simulink model "SimBasZEnvioTodo"  (R2026b)
settings: Solver=VariableStepAuto  StopTime=inf
undefined symbols (not defined in the file): heartbeatBytes, Payload, SampleTime
libraries: uavmavlinklib x8, simulink x1, sharedtransform x1
settings Model: Creator=cfmm  LastModifiedBy=cfmm

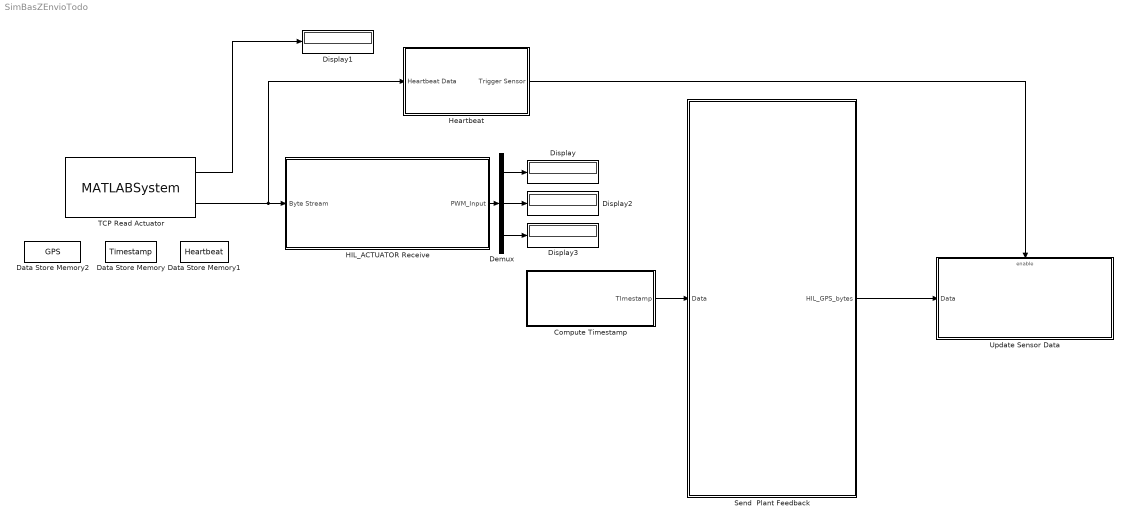
== system SimBasZEnvioTodo ==
  Compute Timestamp : Subsystem
  Data Store Memory : DataStoreMemory  DataStoreName=Timestamp  WriteAfterWriteMsg=warning  ShowAdditionalParam=off
  Data Store Memory1 : DataStoreMemory  DataStoreName=Heartbeat  WriteAfterWriteMsg=warning  InitialValue=1  ShowAdditionalParam=off
  Data Store Memory2 : DataStoreMemory  DataStoreName=GPS  WriteAfterWriteMsg=warning  ShowAdditionalParam=off
  Demux : Demux  Outputs=3
  Display{,1..3} (4 alike) : Display
  HIL_ACTUATOR Receive : Subsystem
  Heartbeat : Subsystem
  Send  Plant Feedback : Subsystem
  TCP Read Actuator : MATLABSystem  System=px4HostTarget_TCPIP_Read  Length=actuatorBytes  SampleTime=SampleTime
      mask Type: px4HostTarget_TCPIP_Read
  "Update Sensor Data " : Subsystem
  wires:
  TCP Read Actuator/1 -> Display1/1
  TCP Read Actuator/2 -> Heartbeat/1(Heartbeat Data), HIL_ACTUATOR Receive/1(Byte Stream)
  Send  Plant Feedback/1(HIL_GPS_bytes) -> "Update Sensor Data "/1(Data)
  Heartbeat/1(Trigger Sensor) -> "Update Sensor Data "/Enable
  HIL_ACTUATOR Receive/1(PWM_Input) -> Demux/1
  Demux/1 -> Display/1
  Demux/2 -> Display2/1
  Demux/3 -> Display3/1
  Compute Timestamp/1(TImestamp) -> Send  Plant Feedback/1(Data)

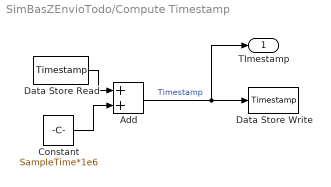
== system SimBasZEnvioTodo/Compute Timestamp ==
  Add : Sum
  Constant : Constant  Value=SampleTime*1e6  OutDataTypeStr=uint64  SampleTime=SampleTime
  Data Store Read : DataStoreRead  DataStoreName=Timestamp  SampleTime=SampleTime  IndexOptions=Index vector (dialog)  Indices=1  OutputSizes=1
  Data Store Write : DataStoreWrite  DataStoreName=Timestamp  SampleTime=SampleTime  IndexOptions=Index vector (dialog)  Indices=1  OutputSizes=1
  TImestamp : Outport
  wires:
  Data Store Read/1 -> Add/1
  Add/1 -> TImestamp/1, Data Store Write/1  "Timestamp"
  Constant/1 -> Add/2

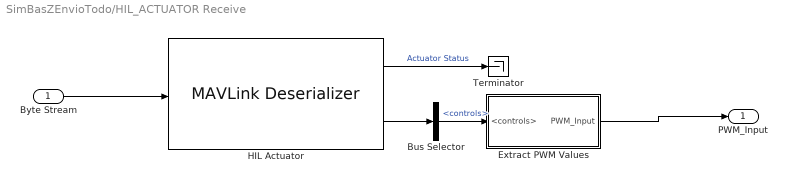
== system SimBasZEnvioTodo/HIL_ACTUATOR Receive ==
  Byte Stream : Inport
  Bus Selector : BusSelector  OutputSignals=Payload.controls
  Extract PWM Values : Subsystem
  HIL Actuator : uavmavlinklib/MAVLink Deserializer  dialectSource=Select from standard MAVLink dialects  dialect=common.xml  dialectCustom=common.xml  version=2  messageType=HIL_ACTUATOR_CONTROLS  inputDataLength=off  SystemIDFilter=off  systemID=1  ComponentIDFilter=off  componentID=1  queueMsg=off  queueMsgSize=50  dropNum=off
  Terminator : Terminator
  PWM_Input : Outport
  wires:
  Byte Stream/1 -> HIL Actuator/1
  HIL Actuator/2 -> Bus Selector/1
  Bus Selector/1 -> Extract PWM Values/1(<controls>)  "<controls>"
  Extract PWM Values/1(PWM_Input) -> PWM_Input/1
  HIL Actuator/1 -> Terminator/1  "Actuator Status"

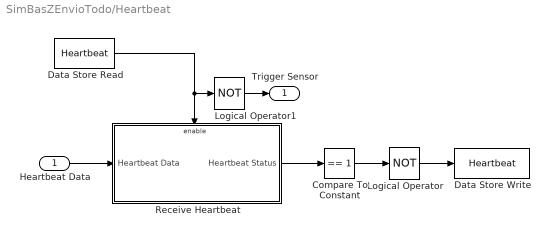
== system SimBasZEnvioTodo/Heartbeat ==
  Heartbeat Data : Inport
  Compare To Constant : simulink/Logic and Bit Operations/Compare To Constant  relop===  const=1  OutDataTypeStr=uint8
  Data Store Read : DataStoreRead  DataStoreName=Heartbeat  SampleTime=SampleTime  IndexOptions=Index vector (dialog)  Indices=1  OutputSizes=1
  Data Store Write : DataStoreWrite  DataStoreName=Heartbeat  SampleTime=SampleTime  IndexOptions=Index vector (dialog)  Indices=1  OutputSizes=1
  Logical Operator : Logic  Operator=NOT  AllPortsSameDT=off  OutDataTypeStr=boolean
  Logical Operator1 : Logic  Operator=NOT  AllPortsSameDT=off  OutDataTypeStr=boolean
  Receive Heartbeat : Subsystem
  Trigger Sensor : Outport
  wires:
  Logical Operator/1 -> Data Store Write/1
  Data Store Read/1 -> Receive Heartbeat/Enable, Logical Operator1/1
  Receive Heartbeat/1(Heartbeat Status) -> Compare To Constant/1
  Compare To Constant/1 -> Logical Operator/1
  Heartbeat Data/1 -> Receive Heartbeat/1(Heartbeat Data)
  Logical Operator1/1 -> Trigger Sensor/1

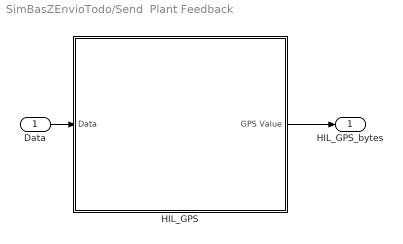
== system SimBasZEnvioTodo/Send  Plant Feedback ==
  Data : Inport
  HIL_GPS : Subsystem
  HIL_GPS_bytes : Outport
  wires:
  HIL_GPS/1(GPS Value) -> HIL_GPS_bytes/1
  Data/1 -> HIL_GPS/1(Data)

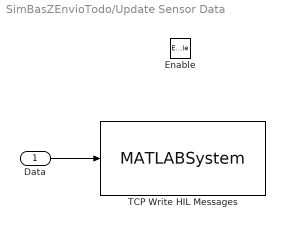
== system SimBasZEnvioTodo/Update Sensor Data  ==
  Data : Inport
  Enable : EnablePort
  TCP Write HIL Messages : MATLABSystem  System=px4HostTarget_TCPIP_Write
      mask Type: px4HostTarget_TCPIP_Write
  wires:
  Data/1 -> TCP Write HIL Messages/1

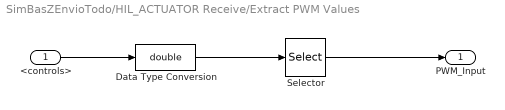
== system SimBasZEnvioTodo/HIL_ACTUATOR Receive/Extract PWM Values ==
  <controls> : Inport
  Data Type Conversion : DataTypeConversion  OutDataTypeStr=double  SaturateOnIntegerOverflow=off  RndMeth=Floor
  Selector : Selector  InputPortWidth=16  IndexOptions=Index vector (dialog)  Indices=[1:3]  OutputSizes=1  RuntimeRangeChecks=off
  PWM_Input : Outport
  wires:
  Data Type Conversion/1 -> Selector/1
  <controls>/1 -> Data Type Conversion/1
  Selector/1 -> PWM_Input/1

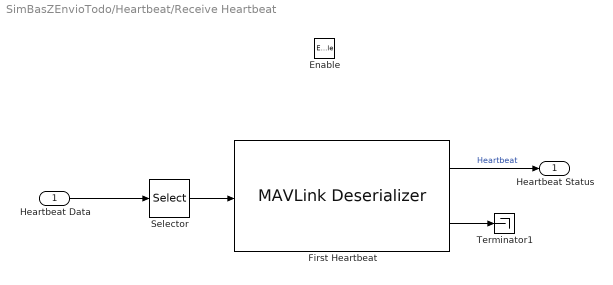
== system SimBasZEnvioTodo/Heartbeat/Receive Heartbeat ==
  Heartbeat Data : Inport
  Enable : EnablePort
  First Heartbeat : uavmavlinklib/MAVLink Deserializer  dialectSource=Select from standard MAVLink dialects  dialect=common.xml  dialectCustom=common.xml  version=2  messageType=HEARTBEAT  inputDataLength=off  SystemIDFilter=off  systemID=1  ComponentIDFilter=off  componentID=1  queueMsg=off  queueMsgSize=50  dropNum=off
  Selector : Selector  InputPortWidth=93  IndexOptions=Index vector (dialog)  Indices=[1:heartbeatBytes]  OutputSizes=1  RuntimeRangeChecks=off
  Terminator1 : Terminator
  Heartbeat Status : Outport
  wires:
  First Heartbeat/2 -> Terminator1/1
  Selector/1 -> First Heartbeat/1
  First Heartbeat/1 -> Heartbeat Status/1  "Heartbeat"
  Heartbeat Data/1 -> Selector/1

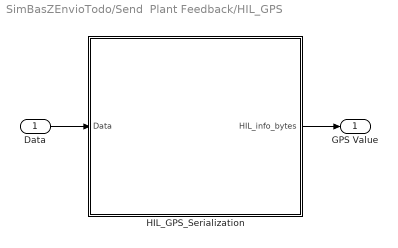
== system SimBasZEnvioTodo/Send  Plant Feedback/HIL_GPS ==
  Data : Inport
  HIL_GPS_Serialization : Subsystem
  GPS Value : Outport
  wires:
  HIL_GPS_Serialization/1(HIL_info_bytes) -> GPS Value/1
  Data/1 -> HIL_GPS_Serialization/1(Data)

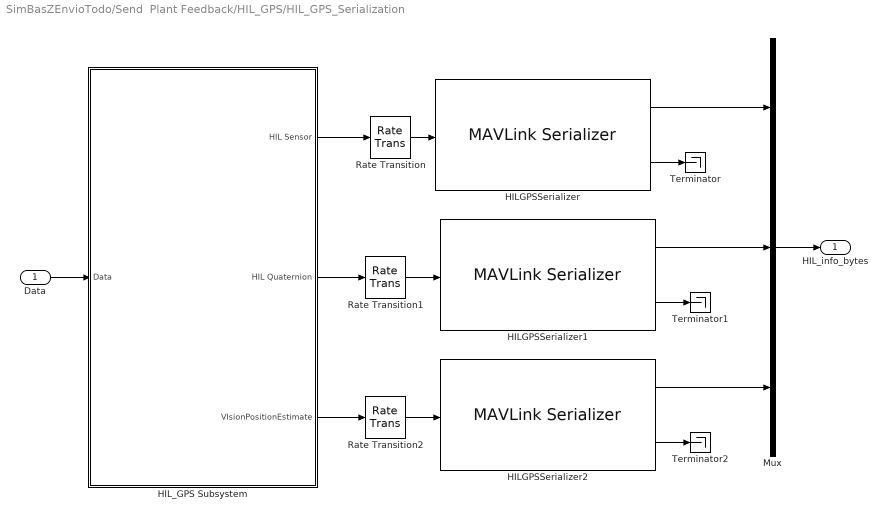
== system SimBasZEnvioTodo/Send  Plant Feedback/HIL_GPS/HIL_GPS_Serialization ==
  Data : Inport
  HILGPSSerializer : uavmavlinklib/MAVLink Serializer  dialectSource=Select from standard MAVLink dialects  dialect=common.xml  dialectCustom=common.xml  version=2  messageType=HIL_SENSOR
  HILGPSSerializer1 : uavmavlinklib/MAVLink Serializer  dialectSource=Select from standard MAVLink dialects  dialect=common.xml  dialectCustom=common.xml  version=2  messageType=HIL_STATE_QUATERNION
  HILGPSSerializer2 : uavmavlinklib/MAVLink Serializer  dialectSource=Select from standard MAVLink dialects  dialect=common.xml  dialectCustom=common.xml  version=2  messageType=VISION_POSITION_ESTIMATE
  HIL_GPS Subsystem : Subsystem
  Mux : Mux  Inputs=3
  Rate Transition : RateTransition  OutPortSampleTime=SampleTime
  Rate Transition1 : RateTransition  OutPortSampleTime=SampleTime
  Rate Transition2 : RateTransition  OutPortSampleTime=SampleTime
  Terminator : Terminator
  Terminator1 : Terminator
  Terminator2 : Terminator
  HIL_info_bytes : Outport
  wires:
  HILGPSSerializer/2 -> Terminator/1
  HIL_GPS Subsystem/1(HIL Sensor) -> Rate Transition/1
  Rate Transition/1 -> HILGPSSerializer/1
  Rate Transition1/1 -> HILGPSSerializer1/1
  HILGPSSerializer1/2 -> Terminator1/1
  HILGPSSerializer2/1 -> Mux/3
  Rate Transition2/1 -> HILGPSSerializer2/1
  HILGPSSerializer2/2 -> Terminator2/1
  HIL_GPS Subsystem/2(HIL Quaternion) -> Rate Transition1/1
  HIL_GPS Subsystem/3(VIsionPositionEstimate) -> Rate Transition2/1
  HILGPSSerializer/1 -> Mux/1
  HILGPSSerializer1/1 -> Mux/2
  Mux/1 -> HIL_info_bytes/1
  Data/1 -> HIL_GPS Subsystem/1(Data)

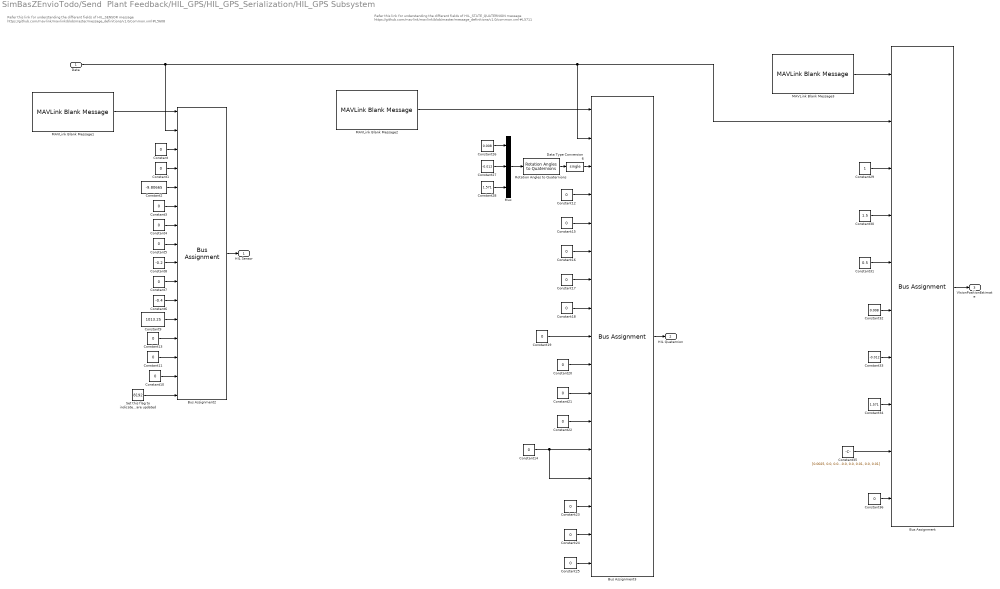
== system SimBasZEnvioTodo/Send  Plant Feedback/HIL_GPS/HIL_GPS_Serialization/HIL_GPS Subsystem ==
  note: Refer this link for understanding the different fields of HIL_SENSOR message https://github.com/mavlink/mavlink/blob/master/message_definitions/v1.0/common.xml#L5608
  note: Refer this link for understanding the different fields of HIL_STATE_QUATERNION message https://github.com/mavlink/mavlink/blob/master/message_definitions/v1.0/common.xml#L5711
  Data : Inport
  Bus Assignment : BusAssignment  AssignedSignals=Payload.usec,Payload.x,Payload.y,Payload.z,Payload.roll,Payload.pitch,Payload.yaw,Payload.covariance,Payload.reset_counter
  Bus Assignment2 : BusAssignment  AssignedSignals=Payload.time_usec,Payload.xacc,Payload.yacc,Payload.zacc,Payload.xgyro,Payload.ygyro,Payload.zgyro,Payload.xmag,Payload.ymag,Payload.zmag,Payload.abs_pressure,Payload.diff_pressure,Payload.pressure_alt,Payload.temperature,Payload.fields_updated
  Bus Assignment3 : BusAssignment  AssignedSignals=Payload.time_usec,Payload.attitude_quaternion,Payload.rollspeed,Payload.pitchspeed,Payload.yawspeed,Payload.lat,Payload.lon,Payload.alt,Payload.vx,Payload.vy,Payload.vz,Payload.ind_airspeed,Payload.true_airspeed,Payload.xacc,Payload.yacc,Payload.zacc
  Constant{,1,3..5,7} (6 alike) : Constant  Value=0  OutDataTypeStr=single
  Constant{10..13,15..16} (6 alike) : Constant  Value=0  OutDataTypeStr=single  SampleTime=SampleTime
  Constant14 : Constant  Value=0  OutDataTypeStr=Inherit: Inherit via back propagation
  Constant17 : Constant  Value=0  OutDataTypeStr=int32  SampleTime=SampleTime
  Constant18 : Constant  Value=0  OutDataTypeStr=int32  SampleTime=SampleTime
  Constant19 : Constant  Value=0  OutDataTypeStr=int32  SampleTime=SampleTime
  Constant2 : Constant  Value=-9.80665  OutDataTypeStr=single
  Constant{20..25} (6 alike) : Constant  Value=0  OutDataTypeStr=int16  SampleTime=SampleTime
  Constant26 : Constant  Value=0.008  OutDataTypeStr=single  SampleTime=SampleTime
  Constant27 : Constant  Value=-0.012  OutDataTypeStr=single  SampleTime=SampleTime
  Constant28 : Constant  Value=1.571  OutDataTypeStr=single  SampleTime=SampleTime
  Constant29 : Constant  OutDataTypeStr=single  SampleTime=SampleTime
  Constant30 : Constant  Value=1.5  OutDataTypeStr=single  SampleTime=SampleTime
  Constant31 : Constant  Value=0.5  OutDataTypeStr=single  SampleTime=SampleTime
  Constant32 : Constant  Value=0.008  OutDataTypeStr=single  SampleTime=SampleTime
  Constant33 : Constant  Value=-0.012  OutDataTypeStr=single  SampleTime=SampleTime
  Constant34 : Constant  Value=1.571  OutDataTypeStr=single  SampleTime=SampleTime
  Constant35 : Constant  Value=[0.0025, 0.0, 0.0, 0.0, 0.0, 0.0, 0.0025, 0.0, 0.0, 0.0, 0.0, 0.0025, 0.0, 0.0, 0.0, 0.01, 0.0, 0.0, 0.01, 0.0, 0.01]  OutDataTypeStr=single  SampleTime=SampleTime
  Constant36 : Constant  Value=0  OutDataTypeStr=uint8  SampleTime=SampleTime
  Constant6 : Constant  Value=-0.4  OutDataTypeStr=single
  Constant8 : Constant  Value=-0.2  OutDataTypeStr=single
  Constant9 : Constant  Value=1013.25  OutDataTypeStr=single
  Data Type Conversion6 : DataTypeConversion  OutDataTypeStr=single  SaturateOnIntegerOverflow=off  RndMeth=Floor
  MAVLink Blank Message1 : uavmavlinklib/MAVLink Blank Message  dialectSource=Select from standard MAVLink dialects  dialect=common.xml  dialectCustom=common.xml  version=2  messageType=HIL_SENSOR  SystemID=2  ComponentID=51  SampleTime=SampleTime
  MAVLink Blank Message2 : uavmavlinklib/MAVLink Blank Message  dialectSource=Select from standard MAVLink dialects  dialect=common.xml  dialectCustom=common.xml  version=2  messageType=HIL_STATE_QUATERNION  SystemID=2  ComponentID=51  SampleTime=SampleTime
  MAVLink Blank Message3 : uavmavlinklib/MAVLink Blank Message  dialectSource=Select from standard MAVLink dialects  dialect=common.xml  dialectCustom=common.xml  version=2  messageType=VISION_POSITION_ESTIMATE  SystemID=2  ComponentID=51  SampleTime=SampleTime
  Mux : Mux  Inputs=3
  Rotation Angles to Quaternions : sharedtransform/Rotation Angles to Quaternions  rotationOrder=ZYX  aMode=aMode
  Set this flag to indicate all flags are updated : Constant  Value=8192  OutDataTypeStr=Inherit: Inherit via back propagation  SampleTime=SampleTime
  HIL Sensor : Outport
  HIL Quaternion : Outport  Port=2
  VIsionPositionEstimate : Outport  Port=3
  wires:
  MAVLink Blank Message1/1 -> Bus Assignment2/1
  Set this flag to indicate all flags are updated/1 -> Bus Assignment2/16
  Bus Assignment2/1 -> HIL Sensor/1
  Constant13/1 -> Bus Assignment2/13
  MAVLink Blank Message2/1 -> Bus Assignment3/1
  Constant14/1 -> Bus Assignment3/14, Bus Assignment3/13
  Rotation Angles to Quaternions/1 -> Data Type Conversion6/1
  Data Type Conversion6/1 -> Bus Assignment3/3
  Bus Assignment3/1 -> HIL Quaternion/1
  MAVLink Blank Message3/1 -> Bus Assignment/1
  Bus Assignment/1 -> VIsionPositionEstimate/1
  Constant/1 -> Bus Assignment2/3
  Constant1/1 -> Bus Assignment2/4
  Constant2/1 -> Bus Assignment2/5
  Constant3/1 -> Bus Assignment2/6
  Constant4/1 -> Bus Assignment2/7
  Constant5/1 -> Bus Assignment2/8
  Constant6/1 -> Bus Assignment2/11
  Constant7/1 -> Bus Assignment2/10
  Constant8/1 -> Bus Assignment2/9
  Constant9/1 -> Bus Assignment2/12
  Constant10/1 -> Bus Assignment2/15
  Constant11/1 -> Bus Assignment2/14
  Constant12/1 -> Bus Assignment3/4
  Constant15/1 -> Bus Assignment3/5
  Constant16/1 -> Bus Assignment3/6
  Constant17/1 -> Bus Assignment3/7
  Constant20/1 -> Bus Assignment3/10
  Constant21/1 -> Bus Assignment3/11
  Constant22/1 -> Bus Assignment3/12
  Constant23/1 -> Bus Assignment3/15
  Constant24/1 -> Bus Assignment3/16
  Constant25/1 -> Bus Assignment3/17
  Data/1 -> Bus Assignment/2, Bus Assignment3/2, Bus Assignment2/2
  Mux/1 -> Rotation Angles to Quaternions/1
  Constant26/1 -> Mux/1
  Constant27/1 -> Mux/2
  Constant28/1 -> Mux/3
  Constant29/1 -> Bus Assignment/3
  Constant30/1 -> Bus Assignment/4
  Constant31/1 -> Bus Assignment/5
  Constant32/1 -> Bus Assignment/6
  Constant33/1 -> Bus Assignment/7
  Constant34/1 -> Bus Assignment/8
  Constant35/1 -> Bus Assignment/9
  Constant36/1 -> Bus Assignment/10
  Constant18/1 -> Bus Assignment3/8
  Constant19/1 -> Bus Assignment3/9
